simulink model "OFDMmodel_synch"  (R2025b)
settings: Solver=VariableStepAuto  StartTime=0.0  StopTime=inf  RelTol=1e-3
values from neighbouring files (symbols this model uses):
  BandasG = NFFT/4-4    (= 12)    [InitOFDM.m]
  Carriers = 1:NFFT    [InitOFDM.m]
  CP = 16    [InitOFDM.m]    (also in OFDMwideband_BEM2D.m = 32)
  DataCarrierIn = Carriers    [InitOFDM.m]
  DataCarriers = numel(DataCarrierIn)    [InitOFDM.m]
  DataCarriersFrame = DataCarriers*FrameSize    [InitOFDM.m]
  FrameSize = 40    [InitOFDM.m]
  FrameTime = Tsymbol*(FrameSize+2)    (= 0.000168)    [InitOFDM.m]
  NFFT = 64    [InitOFDM.m]    (also in OFDMwideband_BEM2D.m = 256)
  pilots = randsrc(numel(PilotIndex),1,[-1 1 1i 1i])*.71    [InitOFDM.m]
  PreambuloFrec = zeros(64,1)    [InitOFDM.m]    (also in Preambulo.mat = [0 0 0 0 0 0 0 0 4 0 0 0 ... (64 elements, 64x1)])
  Ts = 1/Fs    (= 5e-08)    [InitOFDM.m]    (also in OFDMwideband_BEM2D.m = 1e-07)
undefined symbols (not defined in the file or in its folder): ifftshift, j, jet, LogicIndex, Low, magnitude
libraries: simulink x9, dspsigops x7, dspxfrm3 x4, commrflib2 x3, dspswit3 x3, commchan3 x1, commofdm x1, dspobslib x1, dspmathops x1, commrandsrc3 x1, commdigbbndam3 x1
settings Model: PacingRate=0.001000  Creator=Fernando  LastModifiedBy=kutsari
settings SolverCC: AlgebraicLoopSolver=TrustRegion
settings DataIOCC: LimitDataPoints=on  MaxDataPoints=1  DSMLogging=off  SaveTime=off
settings DebuggingCC: SignalRangeChecking=warning  UnconnectedInputMsg=warning  UnconnectedOutputMsg=warning  UnconnectedLineMsg=warning  ArithmeticOperatorsInVariantConditions=warning
settings ModelReferenceCC: EnableRefExpFcnMdlSchedulingChecks=on
settings SFSimCC: CustomCodeUndefinedFunction=UseInterfaceOnly
settings RTWCC: GPUComputeCapability=3.5  DLArmComputeVersion=19.05

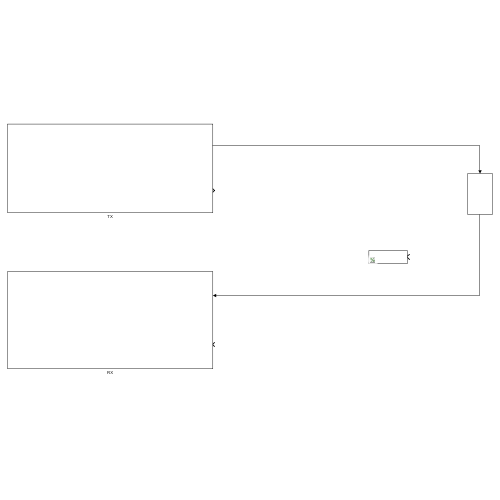
[thumbnail: Simulink's stored preview of the top-level diagram]
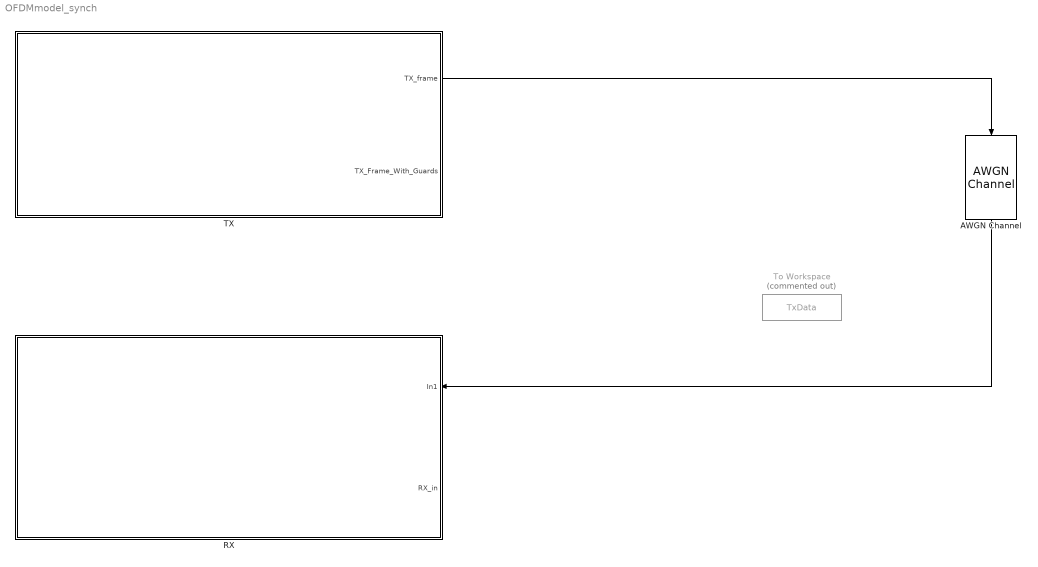
== system OFDMmodel_synch ==
  AWGN Channel : commchan3/AWGN Channel  LegacyMode=on  NoiseMethod="Signal to noise ratio  (SNR)"  noiseMode="Signal to noise ratio  (SNR)"  EbNo=10  EsNo=10  SNR=SNRdb  BitsPerSymbol=1  SignalPower=1  SpecifySymbolPeriod=off  SamplesPerSymbol=1  SymbolPeriod=1  VarianceSource=Parameter  Variance=1  RandomStream=Global stream  Seed=67  SimulateUsing=Code generation
  RX : Subsystem
  TX : Subsystem
  To Workspace : ToWorkspace  Commented=on  VariableName=TxData  SampleTime=-1
  wires:
  AWGN Channel/1 -> RX/1(In1)
  TX/1(TX_frame) -> AWGN Channel/1

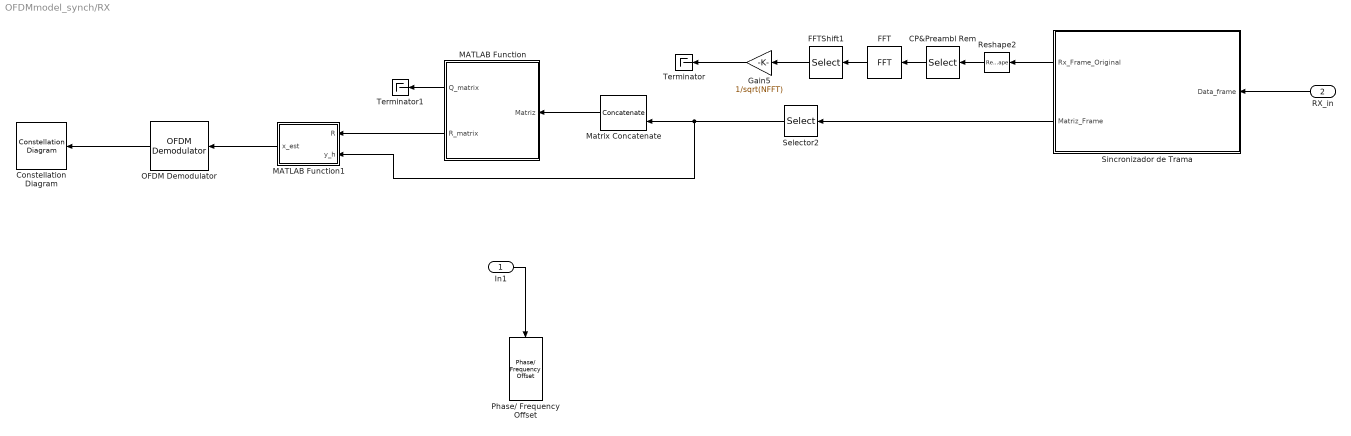
== system OFDMmodel_synch/RX ==
  In1 : Inport
  RX_in : Inport  Port=2
  CP&Preambl Rem : Selector  NumberOfDimensions=2  InputPortWidth=NFFT+CP  IndexOptions=Starting index (dialog),Starting index (dialog)  Indices=CP+1,2  OutputSizes=NFFT,FrameSize
  Constellation Diagram : ConstellationDiagram  DefaultConfigurationName=comm.scopes.ConstellationDiagramBlockCfg
  FFT : dspxfrm3/FFT  FFTImplementation=Auto  CompMethod=Table lookup  TableOpt=NEW  TableOptActive=Speed  BitRevOrder=off  Normalize=off  InheritFFTLength=on  FFTLength=64  WrapInput=on  roundingMode=Floor  overflowMode=off  firstCoeffDataTypeStr=Inherit: Same word length as input  firstCoeffLastDataTypeStr=Inherit: Same word length as input  outputMin=[]  outputMax=[]
  FFTShift1 : Selector  NumberOfDimensions=2  InputPortWidth=NFFT  IndexOptions=Index vector (dialog),Select all  Indices=ifftshift(Carriers),1  OutputSizes=1,1
  Gain5 : Gain  Gain=1/sqrt(NFFT)
  MATLAB Function : MATLAB Function  TreatAsAtomicUnit=on
  MATLAB Function1 : MATLAB Function  TreatAsAtomicUnit=on
  Matrix Concatenate : Concatenate  Mode=Multidimensional array  ConcatenateDimension=2
  OFDM Demodulator : commofdm/OFDM Demodulator  StatePerturbationForJacobian=1.0e-05  FFTLength=64  NumGuardBandCarriers=[6; 5]  RemoveDCCarrier=off  PilotOutputPort=off  PilotCarrierIndices=[12; 26; 40; 54]  CyclicPrefixLength=16  OversamplingFactor=1  NumSymbols=1  NumReceiveAntennas=1  SimulateUsing=Interpreted execution
  Phase/ Frequency Offset : commrflib2/Phase// Frequency Offset  phaseOffset=0  freqPort=off  freqOffset=5e3
  Reshape2 : Reshape  OutputDimensionality=Customize  OutputDimensions=[NFFT+CP,FrameSize+2]
  Selector2 : Selector  NumberOfDimensions=2  InputPortWidth=NFFT  IndexOptions=Index vector (dialog),Index vector (dialog)  Indices=DataCarrierIn,1  OutputSizes=1,1
  Sincronizador de Trama : Subsystem
  Terminator : Terminator
  Terminator1 : Terminator
  wires:
  Selector2/1 -> MATLAB Function1/2(y_h), Matrix Concatenate/2
  FFT/1 -> FFTShift1/1
  Sincronizador de Trama/2(Matriz_Frame) -> Selector2/1
  FFTShift1/1 -> Gain5/1
  Matrix Concatenate/1 -> MATLAB Function/1(Matriz)
  Reshape2/1 -> CP&Preambl Rem/1
  In1/1 -> Phase/ Frequency Offset/1
  Sincronizador de Trama/1(Rx_Frame_Original) -> Reshape2/1
  Gain5/1 -> Terminator/1
  MATLAB Function/1(Q_matrix) -> Terminator1/1
  CP&Preambl Rem/1 -> FFT/1
  MATLAB Function/2(R_matrix) -> MATLAB Function1/1(R)
  MATLAB Function1/1(x_est) -> OFDM Demodulator/1
  OFDM Demodulator/1 -> Constellation Diagram/1
  RX_in/1 -> Sincronizador de Trama/1(Data_frame)

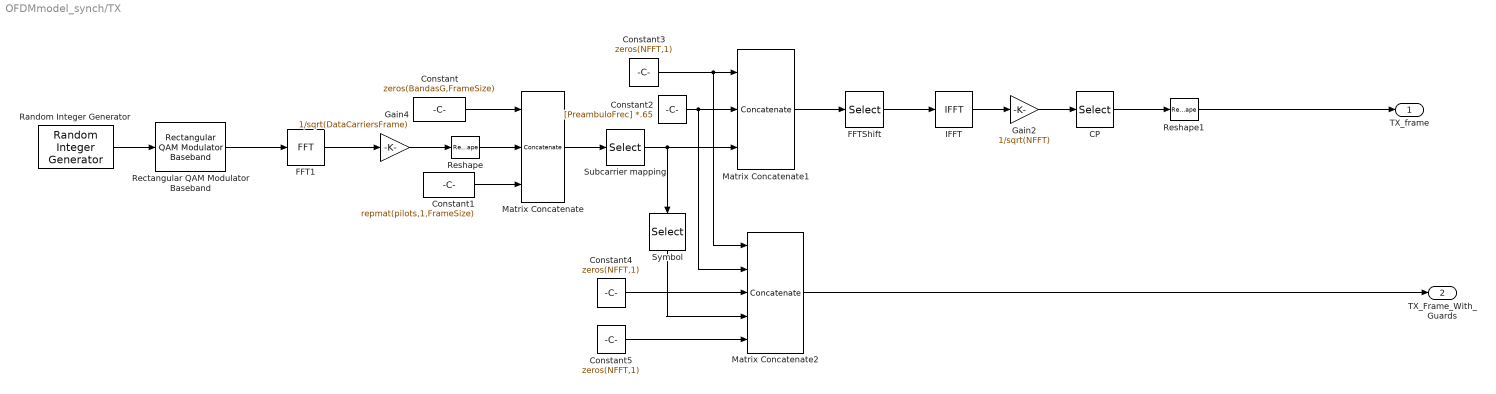
== system OFDMmodel_synch/TX ==
  CP : Selector  NumberOfDimensions=2  InputPortWidth=NFFT  IndexOptions=Index vector (dialog),Select all  Indices=[NFFT-CP+1:NFFT 1:NFFT],1  OutputSizes=1,1
  Constant : Constant  Value=zeros(BandasG,FrameSize)  VectorParams1D=off
  Constant1 : Constant  Value=repmat(pilots,1,FrameSize)  VectorParams1D=off
  Constant2 : Constant  Value=[PreambuloFrec] *.65  VectorParams1D=off
  Constant3 : Constant  Value=zeros(NFFT,1)  VectorParams1D=off
  Constant4 : Constant  Value=zeros(NFFT,1)  VectorParams1D=off
  Constant5 : Constant  Value=zeros(NFFT,1)  VectorParams1D=off
  FFT1 : dspxfrm3/FFT  FFTImplementation=Auto  CompMethod=Table lookup  TableOpt=NEW  TableOptActive=Speed  BitRevOrder=off  Normalize=off  InheritFFTLength=on  FFTLength=64  WrapInput=on  roundingMode=Floor  overflowMode=off  firstCoeffDataTypeStr=Inherit: Same word length as input  firstCoeffLastDataTypeStr=Inherit: Same word length as input  outputMin=[]  outputMax=[]
  FFTShift : Selector  NumberOfDimensions=2  InputPortWidth=NFFT  IndexOptions=Index vector (dialog),Select all  Indices=ifftshift(Carriers),1  OutputSizes=1,1
  Gain2 : Gain  Gain=1/sqrt(NFFT)
  Gain4 : Gain  Gain=1/sqrt(DataCarriersFrame)
  IFFT : dspxfrm3/IFFT  FFTImplementation=Auto  CompMethod=Table lookup  TableOpt=NEW  TableOptActive=Speed  BitRevOrder=off  cs_in=off  Normalize=off  InheritFFTLength=on  FFTLength=64  WrapInput=on  mode=Complex  outSamplingMode=Sample based  roundingMode=Floor  overflowMode=off  firstCoeffDataTypeStr=Inherit: Same word length as input  firstCoeffLastDataTypeStr=Inherit: Same word length as input  outputMin=[]  outputMax=[]
  Matrix Concatenate : Concatenate  NumInputs=3  Mode=Multidimensional array
  Matrix Concatenate1 : Concatenate  NumInputs=3  Mode=Multidimensional array  ConcatenateDimension=2
  Matrix Concatenate2 : Concatenate  NumInputs=5  Mode=Multidimensional array  ConcatenateDimension=2
  Random Integer Generator : commrandsrc3/Random Integer Generator  SetSize=ConstSize  SeedSource=Auto  Seed=0  SampleTime=FrameTime/(DataCarriers*FrameSize)  SamplesPerFrame=DataCarriers*FrameSize  OutputDataType=double  SimulateUsing=Interpreted execution
  Rectangular QAM Modulator Baseband : commdigbbndam3/Rectangular QAM Modulator Baseband  M=ConstSize  InType=Integer  Enc=Gray  Mapping=[0:15]  PowType=Average Power  MinDist=2  AvgPow=1  PeakPow=1  Ph=0  outDtype=double  outWordLen=16  outUDDataType=sfix(16)  outFracLenMode=Best precision  outFracLen=15  outDataTypeStr=double  outLastDataTypeStr=double
  Reshape : Reshape  OutputDimensionality=Customize  OutputDimensions=[DataCarriers,FrameSize]
  Reshape1 : Reshape  OutputDimensionality=Column vector (2-D)  OutputDimensions=[DataCarriers,FrameSize]
  Subcarrier mapping : Selector  NumberOfDimensions=2  InputPortWidth=NFFT  IndexOptions=Index vector (dialog),Select all  Indices=LogicIndex,1  OutputSizes=1,1
  Symbol : Selector  NumberOfDimensions=2  InputPortWidth=NFFT+CP  IndexOptions=Select all,Starting index (dialog)  Indices=CP+1,2  OutputSizes=NFFT,FrameSize-2
  TX_frame : Outport
  TX_Frame_With_Guards : Outport  Port=2
  wires:
  Rectangular QAM Modulator Baseband/1 -> FFT1/1
  CP/1 -> Reshape1/1
  Constant3/1 -> Matrix Concatenate2/1, Matrix Concatenate1/1
  Matrix Concatenate2/1 -> TX_Frame_With_Guards/1
  Matrix Concatenate/1 -> Subcarrier mapping/1
  Random Integer Generator/1 -> Rectangular QAM Modulator Baseband/1
  IFFT/1 -> Gain2/1
  FFT1/1 -> Gain4/1
  Gain4/1 -> Reshape/1
  Constant2/1 -> Matrix Concatenate2/2, Matrix Concatenate1/2
  Reshape/1 -> Matrix Concatenate/2
  Constant/1 -> Matrix Concatenate/1
  Gain2/1 -> CP/1
  Constant4/1 -> Matrix Concatenate2/3
  Subcarrier mapping/1 -> Matrix Concatenate1/3, Symbol/1
  Constant5/1 -> Matrix Concatenate2/5
  Constant1/1 -> Matrix Concatenate/3
  Symbol/1 -> Matrix Concatenate2/4
  Matrix Concatenate1/1 -> FFTShift/1
  FFTShift/1 -> IFFT/1
  Reshape1/1 -> TX_frame/1

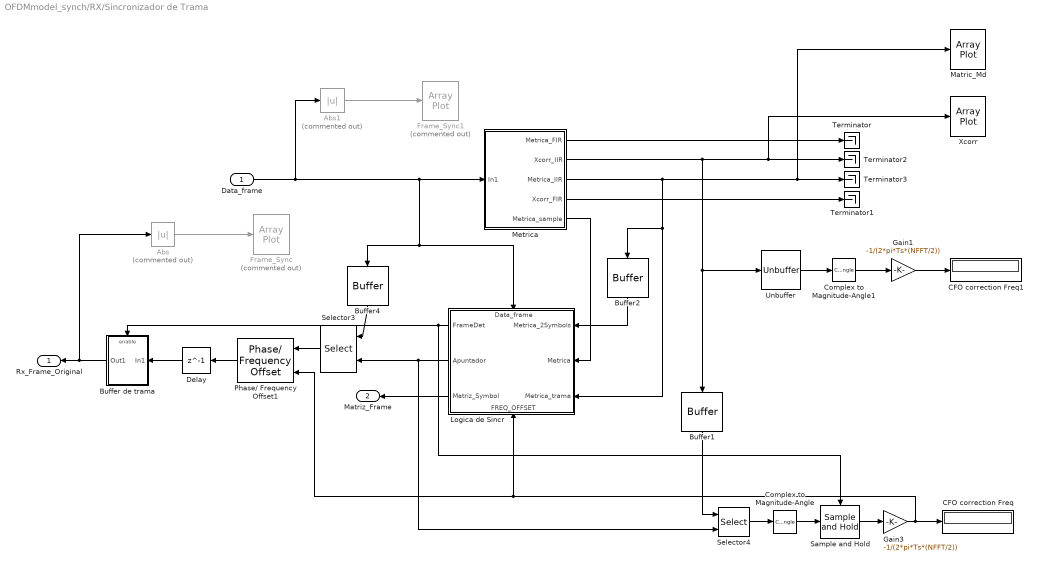
== system OFDMmodel_synch/RX/Sincronizador de Trama ==
  Data_frame : Inport
  Abs : Abs  Commented=on  SaturateOnIntegerOverflow=off
  Abs1 : Abs  Commented=on  SaturateOnIntegerOverflow=off
  Buffer de trama : Subsystem
  Buffer1 : Buffer  N=2*(NFFT+CP)  V=NFFT+CP  OutputFrames=off
  Buffer2 : Buffer  N=2*(NFFT+CP)  V=NFFT+CP  OutputFrames=off
  Buffer4 : Buffer  N=3*(NFFT+CP)  V=2*(NFFT+CP)  OutputFrames=off
  CFO correction Freq : Display
  CFO correction Freq1 : Display
  Complex to Magnitude-Angle : ComplexToMagnitudeAngle  Output=Angle
  Complex to Magnitude-Angle1 : ComplexToMagnitudeAngle  Output=Angle
  Delay : Delay  DelayLength=1
  Frame_Sync : ArrayPlot  Commented=on  WindowPosition=[1 41 1920 963]  AxesScaling=Manual  YLimits=[-0.276842,2.60957]  ShowGrid=off  ChannelNames="[\"\"]"  DefaultConfigurationName=dsp.scopes.ArrayPlotBlockSpecification
  Frame_Sync1 : ArrayPlot  Commented=on  WindowPosition=[1 41 1920 963]  AxesScaling=Manual  YLimits=[-0.026237,2.10871]  ShowGrid=off  ChannelNames="[\"\"]"  DefaultConfigurationName=dsp.scopes.ArrayPlotBlockSpecification
  Gain1 : Gain  Gain=-1/(2*pi*Ts*(NFFT/2))
  Gain3 : Gain  Gain=-1/(2*pi*Ts*(NFFT/2))
  Logica de Sincr : Subsystem
      settings: PortSchema="{\"entries\":[{\"content\":{\"sides\":[{\"content\":{\"connectorIds\":[\"In1\",\"In2\",\"In3\"]},\"type\":\"ConnectorPlacement.EquallySpacedRectSide\",\"uuid\":\"5f8267a0-6860-401f-8e05-bbfffcd5964b\"},{\"content\":{\"connectorIds\":[\"Out1\",\"Out2\",\"Out3\"],\"side\":\"RIGHT\"},\"type\":\"ConnectorPlacement.EquallySpacedRectSide\",\"uuid\":\"fea28aec-daf6-4e63-9655-5b68affc5124\"},{\"content\":{\"connectorIds\":[\"In4\"],\"side\":\"TOP\"},\"type\":\"ConnectorPlacement.EquallySpacedRectSide\",\"uuid\":\"72f5d6e1-ce9a-4296-9270-866e7a0a9494\"},{\"content\":{\"connectorIds\":[\"In5\"],\"side\":\"BOTTOM\"},\"type\":\"ConnectorPlacement.EquallySpacedRectSide\",\"uuid\":\"1736f37f-6e2b-4d11-abf7-aeb554299ece\"},{\"content\":{\"connectorIds\":[],\"side\":\"HIDDEN\"},\"type\":\"ConnectorPlacement.EquallySpacedRectSide\",\"uuid\":\"c53868b6-b813-45ed-ac94-1581b09a364c\"}]},\"type\":\"ConnectorPlacement.EquallySpacedConnector\",\"uuid\":\"ad7f4edf-12d2-4e3f-b534-0670d62195e0\"}],\"packageUris\":[\"http://schema.mathworks.com/mf0/Connector/R2020b\"],\"version\":\"1.0\"}"
  Matric_Md : ArrayPlot  WindowPosition=[481 42 958 954]  AxesScaling=Manual  YLimits=[-0.125,1.125]  ShowGrid=off  ChannelNames="[\"\"]"  DefaultConfigurationName=dsp.scopes.ArrayPlotBlockSpecification
  Metrica : Subsystem
  Phase/ Frequency Offset1 : commrflib2/Phase// Frequency Offset  phaseOffset=0  freqPort=on  freqOffset=16e3
  Sample and Hold : dspsigops/Sample and Hold  trig=Rising edge  initCond=0  latchinput=off
  Selector3 : Selector  InputPortWidth=3*(NFFT+CP)  IndexOptions=Starting index (port)  Indices=[1 3]  OutputSizes=NFFT+CP
  Selector4 : Selector  InputPortWidth=2*(NFFT+CP)  IndexOptions=Index vector (port)  Indices=[1 3]  OutputSizes=1
  Terminator{,1..3} (4 alike) : Terminator
  Unbuffer : Unbuffer
  Xcorr : ArrayPlot  WindowPosition=[481 42 958 954]  AxesScaling=Manual  YLimits=[-0.125,1.125]  ShowGrid=off  ChannelNames="[\"\"]"  DefaultConfigurationName=dsp.scopes.ArrayPlotBlockSpecification
  Rx_Frame_Original : Outport
  Matriz_Frame : Outport  Port=2
  wires:
  Phase/ Frequency Offset1/1 -> Delay/1
  Gain3/1 -> Logica de Sincr/5(FREQ_OFFSET), Phase/ Frequency Offset1/2, CFO correction Freq/1
  Buffer1/1 -> Selector4/1
  Logica de Sincr/2(Apuntador) -> Selector4/2, Selector3/2
  Sample and Hold/1 -> Gain3/1
  Logica de Sincr/1(FrameDet) -> Sample and Hold/Trigger, Buffer de trama/Enable
  Buffer4/1 -> Selector3/1
  Buffer2/1 -> Logica de Sincr/1(Metrica_2Symbols)
  Complex to Magnitude-Angle/1 -> Sample and Hold/1
  Selector3/1 -> Phase/ Frequency Offset1/1
  Metrica/2(Xcorr_IIR) -> Buffer1/1, Unbuffer/1, Xcorr/1, Terminator2/1
  Delay/1 -> Buffer de trama/1(In1)
  Selector4/1 -> Complex to Magnitude-Angle/1
  Data_frame/1 -> Abs1/1, Metrica/1(In1), Logica de Sincr/4(Data_frame), Buffer4/1
  Metrica/3(Metrica_IIR) -> Matric_Md/1, Terminator3/1, Buffer2/1, Logica de Sincr/3(Metrica_trama)
  Buffer de trama/1(Out1) -> Abs/1, Rx_Frame_Original/1
  Metrica/1(Metrica_FIR) -> Terminator/1
  Metrica/5(Metrica_sample) -> Logica de Sincr/2(Metrica)
  Abs/1 -> Frame_Sync/1
  Abs1/1 -> Frame_Sync1/1
  Logica de Sincr/3(Matriz_Symbol) -> Matriz_Frame/1
  Complex to Magnitude-Angle1/1 -> Gain1/1
  Gain1/1 -> CFO correction Freq1/1
  Unbuffer/1 -> Complex to Magnitude-Angle1/1
  Metrica/4(Xcorr_FIR) -> Terminator1/1

== system OFDMmodel_synch/RX/Sincronizador de Trama/Buffer de trama ==
  In1 : Inport
  Enable : EnablePort  ZeroCross=off
  Buffer5 : Buffer  N=(NFFT+CP)*(FrameSize+2)  OutputFrames=off
  Out1 : Outport
  wires:
  In1/1 -> Buffer5/1
  Buffer5/1 -> Out1/1

== system OFDMmodel_synch/RX/Sincronizador de Trama/Logica de Sincr ==
  Metrica_2Symbols : Inport
  Metrica : Inport  Port=2
  Metrica_trama : Inport  Port=3
  Data_frame : Inport  Port=4
  FREQ_OFFSET : Inport  Port=5
  Calculo_indice_Gonzalo_v1 : Subsystem
  Calculo_indice_Gonzalo_v2 : Subsystem
  Calculo_indice_Peña : Subsystem
  Display1 : Display
  Display4 : Display
  Terminator : Terminator
  Terminator1 : Terminator
  FrameDet : Outport
  Apuntador : Outport  Port=2
  Matriz_Symbol : Outport  Port=3
  wires:
  Metrica/1 -> Calculo_indice_Gonzalo_v2/1(Metrica), Calculo_indice_Gonzalo_v1/1(Trigger)
  Data_frame/1 -> Calculo_indice_Gonzalo_v2/2(Data_frame)
  FREQ_OFFSET/1 -> Calculo_indice_Gonzalo_v2/3(Freq_Offset)
  Calculo_indice_Gonzalo_v2/1(Matriz_Symbol) -> Matriz_Symbol/1
  Calculo_indice_Gonzalo_v1/1(Out1) -> Apuntador/1, Display4/1
  Metrica_trama/1 -> Calculo_indice_Gonzalo_v1/2(In2)
  Metrica_2Symbols/1 -> Calculo_indice_Peña/1(In1)
  Calculo_indice_Peña/1(Out1) -> Terminator/1
  Calculo_indice_Peña/2(Out2) -> FrameDet/1
  Calculo_indice_Gonzalo_v2/2(Apuntador_v2) -> Display1/1, Terminator1/1

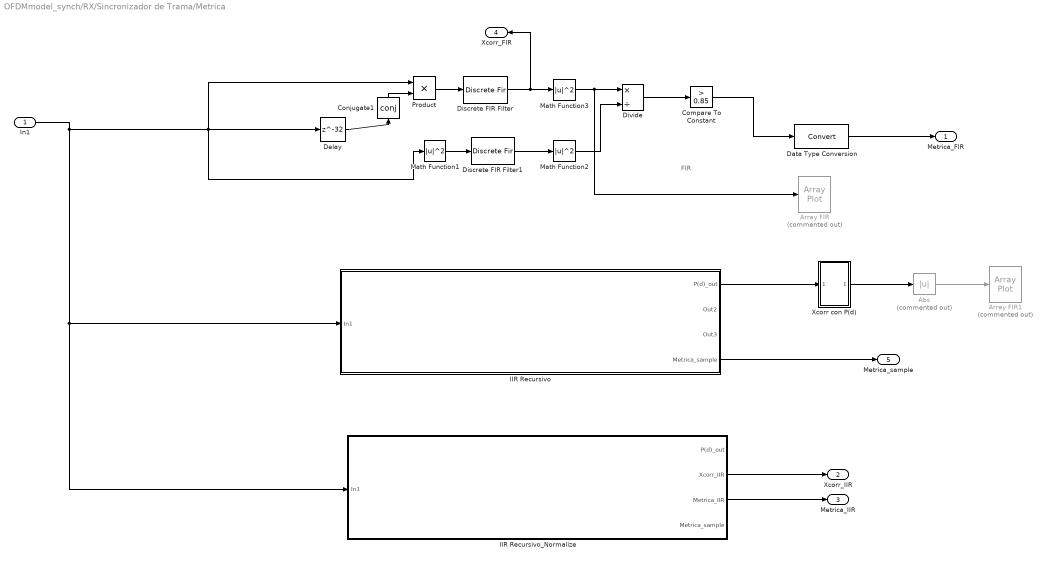
== system OFDMmodel_synch/RX/Sincronizador de Trama/Metrica ==
  note: FIR
  In1 : Inport
  Abs : Abs  Commented=on  SaturateOnIntegerOverflow=off
  Array FIR : ArrayPlot  Commented=on  WindowPosition=[480 -51 958 954]  AxesScaling=Manual  YLimits=[-821.624,7394.62]  ShowGrid=off  ChannelNames="[\"\"]"  DefaultConfigurationName=dsp.scopes.ArrayPlotBlockSpecification
  Array FIR1 : ArrayPlot  Commented=on  WindowPosition=[2 -5 1920 963]  AxesScaling=Manual  YLimits=[-16377.7,109222]  ShowGrid=off  ChannelNames="[\"\"]"  DefaultConfigurationName=dsp.scopes.ArrayPlotBlockSpecification
  Compare To Constant : simulink/Logic and Bit Operations/Compare To Constant  relop=>  const=0.85  OutDataTypeStr=uint8  ZeroCross=off
  Conjugate1 : Math  Operator=conj  SignedPower=on  RndMeth=Zero
  Data Type Conversion : DataTypeConversion  SaturateOnIntegerOverflow=off  RndMeth=Floor
  Delay : Delay  DelayLength=32  InputProcessing=Columns as channels (frame based)
  Discrete FIR Filter : DiscreteFir  Coefficients=ones(1,32)  InputProcessing=Columns as channels (frame based)
  Discrete FIR Filter1 : DiscreteFir  Coefficients=0.5*ones(1,NFFT)  InputProcessing=Columns as channels (frame based)
  Divide : Product  Inputs=*/
  IIR Recursivo : Subsystem
  IIR Recursivo_Normalize : Subsystem
  Math Function1 : Math  Operator=magnitude^2  SignedPower=on
  Math Function2 : Math  Operator=magnitude^2  SignedPower=on
  Math Function3 : Math  Operator=magnitude^2  SignedPower=on
  Product : Product
  Xcorr con P(d) : Subsystem
  Metrica_FIR : Outport
  Xcorr_IIR : Outport  Port=2
  Metrica_IIR : Outport  Port=3
  Xcorr_FIR : Outport  Port=4
  Metrica_sample : Outport  Port=5
  wires:
  Delay/1 -> Conjugate1/1
  Discrete FIR Filter/1 -> Xcorr_FIR/1, Math Function3/1
  Product/1 -> Discrete FIR Filter/1
  Math Function1/1 -> Discrete FIR Filter1/1
  Compare To Constant/1 -> Data Type Conversion/1
  Discrete FIR Filter1/1 -> Math Function2/1
  Math Function3/1 -> Array FIR/1, Divide/1
  Math Function2/1 -> Divide/2
  Data Type Conversion/1 -> Metrica_FIR/1
  Conjugate1/1 -> Product/2
  Divide/1 -> Compare To Constant/1
  In1/1 -> IIR Recursivo_Normalize/1(In1), IIR Recursivo/1(In1), Product/1, Delay/1, Math Function1/1
  IIR Recursivo/1(P(d)_out) -> Xcorr con P(d)/1(In1)
  Xcorr con P(d)/1(Out1) -> Abs/1
  Abs/1 -> Array FIR1/1
  IIR Recursivo/4(Metrica_sample) -> Metrica_sample/1
  IIR Recursivo_Normalize/2(Xcorr_IIR) -> Xcorr_IIR/1
  IIR Recursivo_Normalize/3(Metrica_IIR) -> Metrica_IIR/1

== system OFDMmodel_synch/RX/Sincronizador de Trama/Logica de Sincr/Calculo_indice_Gonzalo_v1 ==
  Trigger : Inport
  In2 : Inport  Port=2
  Bias1 : Bias  Bias=4  SaturateOnIntegerOverflow=off
  Compare To Constant : simulink/Logic and Bit Operations/Compare To Constant  relop=>=  const=NFFT+CP  OutDataTypeStr=boolean
  Display : Display
  Display1 : Display
  Gain : Gain  Gain=1/2
  Gain1 : Gain  Gain=transpose(1:42*(NFFT+CP))
  Rate Transition : RateTransition  OutPortSampleTime=4e-6
  Round1 : Rounding  Operator=round
  Sample and Hold1 : dspsigops/Sample and Hold  trig=Falling edge  initCond=0  latchinput=off
  Sample and Hold2 : dspsigops/Sample and Hold  trig=Rising edge  initCond=0  latchinput=off
  Sample and Hold3 : dspsigops/Sample and Hold  trig=Rising edge  initCond=0  latchinput=off
  Saturation1 : Saturate  UpperLimit=2*(NFFT+CP)+1  LowerLimit=1
  Sum2 : Sum
  Unbuffer : Unbuffer
  Out1 : Outport
  wires:
  Unbuffer/1 -> Sample and Hold1/1, Sample and Hold2/1
  Sample and Hold1/1 -> Sum2/2, Display1/1
  Sample and Hold2/1 -> Sum2/1, Display/1
  Gain/1 -> Round1/1
  Sample and Hold3/1 -> Bias1/1
  Compare To Constant/1 -> Sample and Hold3/Trigger
  Bias1/1 -> Saturation1/1
  Sum2/1 -> Gain/1
  Saturation1/1 -> Rate Transition/1
  Trigger/1 -> Sample and Hold2/Trigger, Sample and Hold1/Trigger
  Round1/1 -> Compare To Constant/1, Sample and Hold3/1
  In2/1 -> Gain1/1
  Gain1/1 -> Unbuffer/1
  Rate Transition/1 -> Out1/1

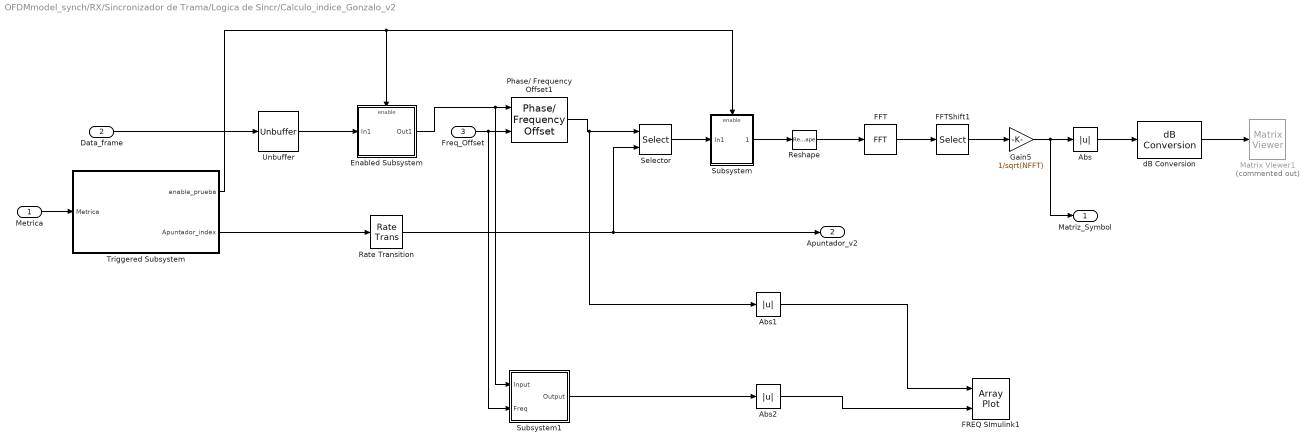
== system OFDMmodel_synch/RX/Sincronizador de Trama/Logica de Sincr/Calculo_indice_Gonzalo_v2 ==
  Metrica : Inport
  Data_frame : Inport  Port=2
  Freq_Offset : Inport  Port=3
  Abs : Abs  SaturateOnIntegerOverflow=off
  Abs1 : Abs  SaturateOnIntegerOverflow=off
  Abs2 : Abs  SaturateOnIntegerOverflow=off
  Enabled Subsystem : Subsystem  TreatAsAtomicUnit=on
  FFT : dspxfrm3/FFT  FFTImplementation=Auto  CompMethod=Table lookup  TableOpt=NEW  TableOptActive=Speed  BitRevOrder=off  Normalize=off  InheritFFTLength=on  FFTLength=64  WrapInput=on  roundingMode=Floor  overflowMode=off  firstCoeffDataTypeStr=Inherit: Same word length as input  firstCoeffLastDataTypeStr=Inherit: Same word length as input  outputMin=[]  outputMax=[]
  FFTShift1 : Selector  NumberOfDimensions=2  InputPortWidth=NFFT  IndexOptions=Index vector (dialog),Select all  Indices=ifftshift(Carriers),1  OutputSizes=1,1
  FREQ SImulink1 : ArrayPlot  NumInputPorts=2  WindowPosition=[99.000000,117.000000,1918.000000,954.000000,]  ScopeFrameLocation=window  AxesScaling=Manual  YLimits=[-0.0514301,1.04318]  ShowGrid=off  ChannelNames="[\"\"]"  DefaultConfigurationName=dsp.scopes.ArrayPlotBlockSpecification
  Gain5 : Gain  Gain=1/sqrt(NFFT)
  Matrix Viewer1 : dspobslib/Matrix Viewer  Commented=on  ImageParams=off  CMapStr=jet(256)  AxisColorbar=on  AxisParams=off  AxisOrigin=Upper left corner  AxisTickMode=Auto  XTickRange=[0 1]  YTickRange=[0 1]  XLabel=X-axis  YLabel=Y-axis  ZLabel=Z-axis  FigPos=[962 42 958 1008]  AxisZoom=off
      settings: YMin=-30  YMax=-20
  Phase/ Frequency Offset1 : commrflib2/Phase// Frequency Offset  phaseOffset=0  freqPort=on  freqOffset=16e3
  Rate Transition : RateTransition  OutPortSampleTime=4e-6
  Reshape : Reshape  OutputDimensionality=Customize  OutputDimensions=[(NFFT),40]
  Selector : Selector  InputPortWidth=NFFT+CP  IndexOptions=Starting index (port)  Indices=[1 3]  OutputSizes=NFFT
  Subsystem : Subsystem
  Subsystem1 : Subsystem
  Triggered Subsystem : Subsystem  TreatAsAtomicUnit=on
  Unbuffer : Unbuffer
  dB Conversion : dspmathops/dB Conversion  dBtype=dB  intype=Amplitude  R=1  fuzz=off
  Matriz_Symbol : Outport
  Apuntador_v2 : Outport  Port=2
  wires:
  Metrica/1 -> Triggered Subsystem/1(Metrica)
  Data_frame/1 -> Unbuffer/1
  Abs/1 -> dB Conversion/1
  Unbuffer/1 -> Enabled Subsystem/1(In1)
  Enabled Subsystem/1(Out1) -> Subsystem1/1(Input), Phase/ Frequency Offset1/1
  Rate Transition/1 -> Selector/2, Apuntador_v2/1
  dB Conversion/1 -> Matrix Viewer1/1
  FFT/1 -> FFTShift1/1
  FFTShift1/1 -> Gain5/1
  Reshape/1 -> FFT/1
  Gain5/1 -> Matriz_Symbol/1, Abs/1
  Subsystem/1(Trama_sin_CP) -> Reshape/1
  Phase/ Frequency Offset1/1 -> Abs1/1, Selector/1
  Freq_Offset/1 -> Subsystem1/2(Freq), Phase/ Frequency Offset1/2
  Selector/1 -> Subsystem/1(In1)
  Triggered Subsystem/2(Apuntador_index) -> Rate Transition/1
  Triggered Subsystem/1(enable_prueba) -> Subsystem/Enable, Enabled Subsystem/Enable
  Subsystem1/1(Output) -> Abs2/1
  Abs1/1 -> FREQ SImulink1/1
  Abs2/1 -> FREQ SImulink1/2

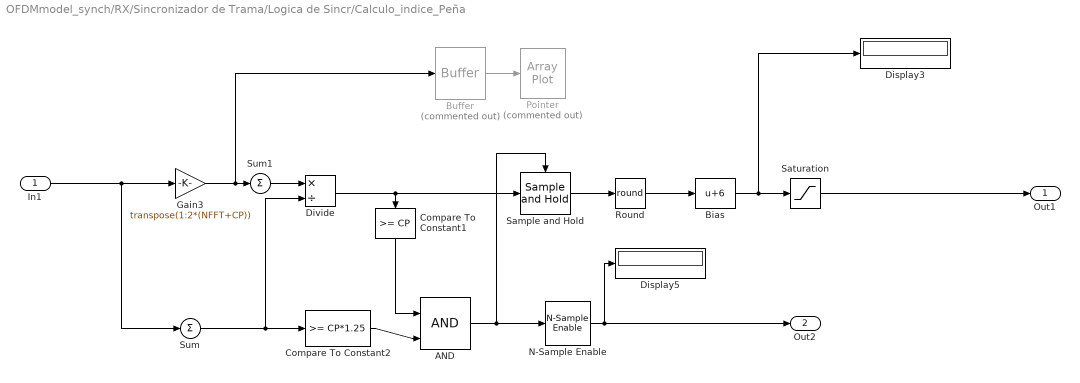
== system OFDMmodel_synch/RX/Sincronizador de Trama/Logica de Sincr/Calculo_indice_Peña ==
  In1 : Inport
  AND : Logic  IconShape=distinctive  AllPortsSameDT=off  OutDataTypeStr=boolean
  Bias : Bias  Bias=6  SaturateOnIntegerOverflow=off
  Buffer : Buffer  Commented=on  N=2*(NFFT + CP)  OutputFrames=off
  Compare To Constant1 : simulink/Logic and Bit Operations/Compare To Constant  relop=>=  const=CP  OutDataTypeStr=boolean  ZeroCross=off
  Compare To Constant2 : simulink/Logic and Bit Operations/Compare To Constant  relop=>=  const=CP*1.25  OutDataTypeStr=boolean  ZeroCross=off
  Display3 : Display
  Display5 : Display
  Divide : Product  Inputs=*/
  Gain3 : Gain  Gain=transpose(1:2*(NFFT+CP))
  N-Sample Enable : dspswit3/N-Sample Enable  N=FrameSize+1  ActiveLevel=Low (0)  reset=on  TriggerType=Rising edge  Ts=1  DataType=Logical
  Pointer : ArrayPlot  Commented=on  WindowPosition=[481 42 958 954]  AxesScaling=Manual  YLimits=[-16.5,168.5]  ShowGrid=off  ChannelNames="[\"\"]"  DefaultConfigurationName=dsp.scopes.ArrayPlotBlockSpecification
  Round : Rounding  Operator=round
  Sample and Hold : dspsigops/Sample and Hold  trig=Rising edge  initCond=0  latchinput=off
  Saturation : Saturate  UpperLimit=2*(NFFT+CP)+1  LowerLimit=1
  Sum : Sum  Inputs=+
  Sum1 : Sum  Inputs=+
  Out1 : Outport
  Out2 : Outport  Port=2
  wires:
  Sum/1 -> Divide/2, Compare To Constant2/1
  Bias/1 -> Display3/1, Saturation/1
  Gain3/1 -> Buffer/1, Sum1/1
  Sample and Hold/1 -> Round/1
  Divide/1 -> Sample and Hold/1, Compare To Constant1/1
  Compare To Constant2/1 -> AND/2
  Buffer/1 -> Pointer/1
  AND/1 -> Sample and Hold/Trigger, N-Sample Enable/1
  In1/1 -> Sum/1, Gain3/1
  N-Sample Enable/1 -> Out2/1, Display5/1
  Round/1 -> Bias/1
  Saturation/1 -> Out1/1
  Sum1/1 -> Divide/1
  Compare To Constant1/1 -> AND/1

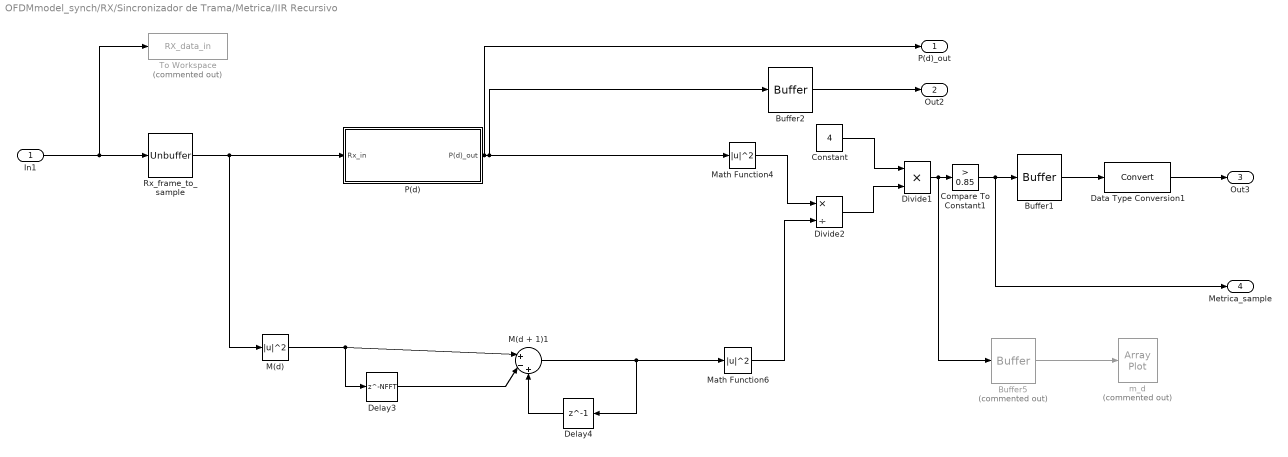
== system OFDMmodel_synch/RX/Sincronizador de Trama/Metrica/IIR Recursivo ==
  In1 : Inport
  Buffer1 : Buffer  N=(NFFT + CP) * 42  OutputFrames=off
  Buffer2 : Buffer  N=(NFFT + CP) * 42  OutputFrames=off
  Buffer5 : Buffer  Commented=on  N=(NFFT + CP) * 42  OutputFrames=off
  Compare To Constant1 : simulink/Logic and Bit Operations/Compare To Constant  relop=>  const=0.85  OutDataTypeStr=uint8  ZeroCross=off
  Constant : Constant  Value=4
  Data Type Conversion1 : DataTypeConversion  SaturateOnIntegerOverflow=off  RndMeth=Floor
  Delay3 : Delay  DelayLength=NFFT
  Delay4 : Delay  DelayLength=1
  Divide1 : Product  Inputs=**
  Divide2 : Product  Inputs=*/
  M(d + 1)1 : Sum  Inputs=|+-+
  M(d) : Math  Operator=magnitude^2  SignedPower=on
  Math Function4 : Math  Operator=magnitude^2  SignedPower=on
  Math Function6 : Math  Operator=magnitude^2  SignedPower=on
  P(d) : Subsystem
  Rx_frame_to_sample : Unbuffer
  To Workspace : ToWorkspace  Commented=on  VariableName=RX_data_in  SaveFormat=Timeseries  SampleTime=-1
  m_d : ArrayPlot  Commented=on  WindowPosition=[1 41 1920 963]  AxesScaling=Manual  YLimits=[-0.116212,1.04604]  ShowGrid=off  ChannelNames="[\"\"]"  DefaultConfigurationName=dsp.scopes.ArrayPlotBlockSpecification
  P(d)_out : Outport
  Out2 : Outport  Port=2
  Out3 : Outport  Port=3
  Metrica_sample : Outport  Port=4
  wires:
  M(d)/1 -> M(d + 1)1/1, Delay3/1
  Delay4/1 -> M(d + 1)1/3
  Buffer1/1 -> Data Type Conversion1/1
  Math Function6/1 -> Divide2/2
  Compare To Constant1/1 -> Metrica_sample/1, Buffer1/1
  Divide2/1 -> Divide1/2
  Divide1/1 -> Buffer5/1, Compare To Constant1/1
  Buffer2/1 -> Out2/1
  Delay3/1 -> M(d + 1)1/2
  Math Function4/1 -> Divide2/1
  Constant/1 -> Divide1/1
  In1/1 -> To Workspace/1, Rx_frame_to_sample/1
  Data Type Conversion1/1 -> Out3/1
  M(d + 1)1/1 -> Math Function6/1, Delay4/1
  Buffer5/1 -> m_d/1
  Rx_frame_to_sample/1 -> P(d)/1(Rx_in), M(d)/1
  P(d)/1(P(d)_out) -> P(d)_out/1, Buffer2/1, Math Function4/1

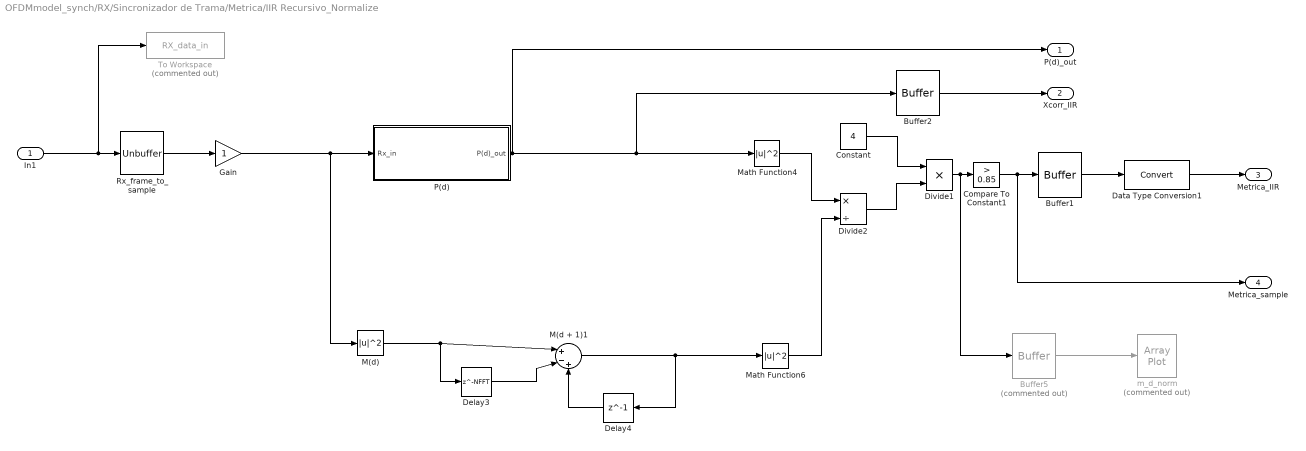
== system OFDMmodel_synch/RX/Sincronizador de Trama/Metrica/IIR Recursivo_Normalize ==
  In1 : Inport
  Buffer1 : Buffer  N=(NFFT + CP) * 42  OutputFrames=off
  Buffer2 : Buffer  N=(NFFT + CP) * 42  OutputFrames=off
  Buffer5 : Buffer  Commented=on  N=(NFFT + CP) * 42  OutputFrames=off
  Compare To Constant1 : simulink/Logic and Bit Operations/Compare To Constant  relop=>  const=0.85  OutDataTypeStr=uint8  ZeroCross=off
  Constant : Constant  Value=4
  Data Type Conversion1 : DataTypeConversion  SaturateOnIntegerOverflow=off  RndMeth=Floor
  Delay3 : Delay  DelayLength=NFFT
  Delay4 : Delay  DelayLength=1
  Divide1 : Product  Inputs=**
  Divide2 : Product  Inputs=*/
  Gain : Gain
  M(d + 1)1 : Sum  Inputs=|+-+
  M(d) : Math  Operator=magnitude^2  SignedPower=on
  Math Function4 : Math  Operator=magnitude^2  SignedPower=on
  Math Function6 : Math  Operator=magnitude^2  SignedPower=on
  P(d) : Subsystem
  Rx_frame_to_sample : Unbuffer
  To Workspace : ToWorkspace  Commented=on  VariableName=RX_data_in  SaveFormat=Timeseries  SampleTime=-1
  m_d_norm : ArrayPlot  Commented=on  WindowPosition=[1 41 1920 963]  AxesScaling=Manual  YLimits=[-0.116212,1.04604]  ShowGrid=off  ChannelNames="[\"\"]"  DefaultConfigurationName=dsp.scopes.ArrayPlotBlockSpecification
  P(d)_out : Outport
  Xcorr_IIR : Outport  Port=2
  Metrica_IIR : Outport  Port=3
  Metrica_sample : Outport  Port=4
  wires:
  P(d)/1(P(d)_out) -> Math Function4/1, Buffer2/1, P(d)_out/1
  Rx_frame_to_sample/1 -> Gain/1
  Buffer5/1 -> m_d_norm/1
  M(d + 1)1/1 -> Delay4/1, Math Function6/1
  Data Type Conversion1/1 -> Metrica_IIR/1
  In1/1 -> Rx_frame_to_sample/1, To Workspace/1
  Constant/1 -> Divide1/1
  Math Function4/1 -> Divide2/1
  Delay3/1 -> M(d + 1)1/2
  Buffer2/1 -> Xcorr_IIR/1
  Divide1/1 -> Compare To Constant1/1, Buffer5/1
  Divide2/1 -> Divide1/2
  Compare To Constant1/1 -> Buffer1/1, Metrica_sample/1
  Math Function6/1 -> Divide2/2
  Buffer1/1 -> Data Type Conversion1/1
  Delay4/1 -> M(d + 1)1/3
  M(d)/1 -> Delay3/1, M(d + 1)1/1
  Gain/1 -> P(d)/1(Rx_in), M(d)/1

== system OFDMmodel_synch/RX/Sincronizador de Trama/Metrica/Xcorr con P(d) ==
  In1 : Inport
  Buffer3 : Buffer  N=(NFFT + CP) * 42  OutputFrames=off
  Conjugate3 : Math  Operator=conj  SignedPower=on  RndMeth=Zero
  Delay1 : Delay  DelayLength=1
  Delay2 : Delay  DelayLength=NFFT/2  InputProcessing=Columns as channels (frame based)
  Delay5 : Delay  DelayLength=NFFT/2  InputProcessing=Columns as channels (frame based)
  P(d + 1) : Sum  Inputs=|+-+
  P(d) : Product
  Out1 : Outport
  wires:
  Conjugate3/1 -> P(d)/2
  P(d)/1 -> Delay2/1, P(d + 1)/1
  Delay2/1 -> P(d + 1)/2
  Delay5/1 -> Conjugate3/1
  Delay1/1 -> P(d + 1)/3
  In1/1 -> P(d)/1, Delay5/1
  Buffer3/1 -> Out1/1
  P(d + 1)/1 -> Delay1/1, Buffer3/1

== system OFDMmodel_synch/RX/Sincronizador de Trama/Logica de Sincr/Calculo_indice_Gonzalo_v2/Enabled Subsystem ==
  In1 : Inport
  Enable : EnablePort
  Buffer : Buffer  N=NFFT + CP  OutputFrames=off
  Out1 : Outport
  wires:
  In1/1 -> Buffer/1
  Buffer/1 -> Out1/1

== system OFDMmodel_synch/RX/Sincronizador de Trama/Logica de Sincr/Calculo_indice_Gonzalo_v2/Subsystem ==
  In1 : Inport
  Enable : EnablePort
  Buffer : Buffer  N=(NFFT) * 40  OutputFrames=off
  Trama_sin_CP : Outport
  wires:
  In1/1 -> Buffer/1
  Buffer/1 -> Trama_sin_CP/1

== system OFDMmodel_synch/RX/Sincronizador de Trama/Logica de Sincr/Calculo_indice_Gonzalo_v2/Subsystem1 ==
  Input : Inport
  Freq : Inport  Port=2
  Cosine : simulink/Lookup Tables/Cosine  Formula=exp(j*2*pi*u)  NumDataPoints=(2^5)+1  OutputWordLength=16  InternalRulePriority=Speed
  Product : Product
  Output : Outport
  wires:
  Freq/1 -> Cosine/1
  Cosine/1 -> Product/2
  Input/1 -> Product/1
  Product/1 -> Output/1

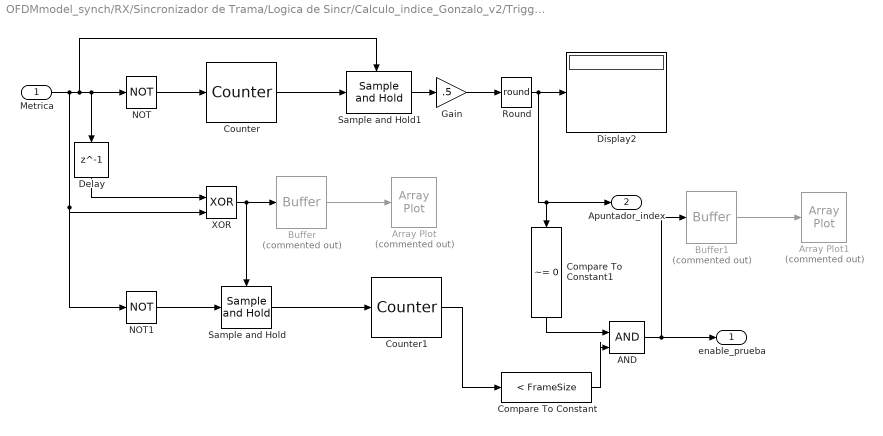
== system OFDMmodel_synch/RX/Sincronizador de Trama/Logica de Sincr/Calculo_indice_Gonzalo_v2/Triggered Subsystem ==
  Metrica : Inport
  AND : Logic  IconShape=distinctive  AllPortsSameDT=off  OutDataTypeStr=boolean
  Array Plot : ArrayPlot  Commented=on  WindowPosition=[2 42 1918 954]  Visible=on  AxesScaling=Manual  YLimits=[-0.0210134,1.03035]  ShowGrid=off  ChannelNames="[\"\"]"  DefaultConfigurationName=dsp.scopes.ArrayPlotBlockSpecification
  Array Plot1 : ArrayPlot  Commented=on  WindowPosition=[-1919 41 1920 963]  AxesScaling=Manual  YLimits=[-0.0584261,0.108841]  ShowGrid=off  ChannelNames="[\"\"]"  DefaultConfigurationName=dsp.scopes.ArrayPlotBlockSpecification
  Buffer : Buffer  Commented=on  N=(80*42)  OutputFrames=off
  Buffer1 : Buffer  Commented=on  N=(80*42)  OutputFrames=off
  Compare To Constant : simulink/Logic and Bit Operations/Compare To Constant  relop=<  const=FrameSize  OutDataTypeStr=boolean
  Compare To Constant1 : simulink/Logic and Bit Operations/Compare To Constant  relop=~=  const=0  OutDataTypeStr=boolean
  Counter : dspswit3/Counter  Direction=Up  CountEvent=Free running  CounterSize=User defined  MaxCount=79  InitialCount=1  Output=Count  HitValue=32  ResetInput=on  SamplesPerFrame=1  Ts=50e-9  CntDtype=double  HitDtype=Logical
  Counter1 : dspswit3/Counter  Direction=Up  CountEvent=Free running  CounterSize=User defined  MaxCount=79  InitialCount=0  Output=Count  HitValue=32  ResetInput=on  SamplesPerFrame=1  Ts=4e-6  CntDtype=double  HitDtype=Logical
  Delay : Delay  DelayLength=1
  Display2 : Display
  Gain : Gain  Gain=.5
  NOT : Logic  Operator=NOT  IconShape=distinctive  AllPortsSameDT=off  OutDataTypeStr=boolean
  NOT1 : Logic  Operator=NOT  IconShape=distinctive  AllPortsSameDT=off  OutDataTypeStr=boolean
  Round : Rounding  Operator=round
  Sample and Hold : dspsigops/Sample and Hold  trig=Rising edge  initCond=1  latchinput=on
  Sample and Hold1 : dspsigops/Sample and Hold  trig=Falling edge  initCond=1  latchinput=on
  XOR : Logic  Operator=XOR  IconShape=distinctive  AllPortsSameDT=off  OutDataTypeStr=boolean
  enable_prueba : Outport
  Apuntador_index : Outport  Port=2
  wires:
  Sample and Hold1/1 -> Gain/1
  Gain/1 -> Round/1
  Counter/1 -> Sample and Hold1/1
  Round/1 -> Compare To Constant1/1, Apuntador_index/1, Display2/1
  Metrica/1 -> NOT1/1, XOR/2, Sample and Hold1/Trigger, NOT/1, Delay/1
  NOT/1 -> Counter/1
  Delay/1 -> XOR/1
  Buffer/1 -> Array Plot/1
  XOR/1 -> Sample and Hold/Trigger, Buffer/1
  Counter1/1 -> Compare To Constant/1
  Sample and Hold/1 -> Counter1/1
  NOT1/1 -> Sample and Hold/1
  AND/1 -> Buffer1/1, enable_prueba/1
  Compare To Constant/1 -> AND/2
  Compare To Constant1/1 -> AND/1
  Buffer1/1 -> Array Plot1/1

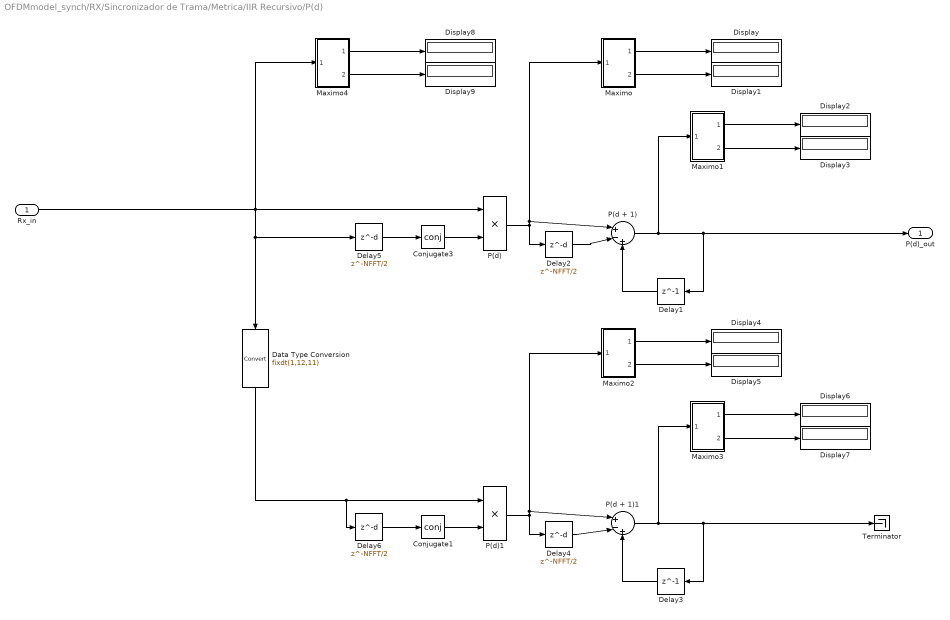
== system OFDMmodel_synch/RX/Sincronizador de Trama/Metrica/IIR Recursivo/P(d) ==
  Rx_in : Inport
  Conjugate1 : Math  Operator=conj  SignedPower=on  RndMeth=Zero
  Conjugate3 : Math  Operator=conj  SignedPower=on  RndMeth=Zero
  Data Type Conversion : DataTypeConversion  OutDataTypeStr=fixdt(1,12,11)  SaturateOnIntegerOverflow=off  RndMeth=Floor  LockScale=on
  Delay1 : Delay  DelayLength=1
  Delay{2,4..6} (4 alike) : Delay  DelayLength=NFFT/2  InputProcessing=Columns as channels (frame based)
  Delay3 : Delay  DelayLength=1
  Display{,1..9} (10 alike) : Display
  Maximo : Subsystem
  Maximo1 : Subsystem
  Maximo2 : Subsystem
  Maximo3 : Subsystem
  Maximo4 : Subsystem
  P(d + 1) : Sum  Inputs=|+-+
  P(d + 1)1 : Sum  Inputs=|+-+
  P(d) : Product
  P(d)1 : Product
  Terminator : Terminator
  P(d)_out : Outport
  wires:
  Delay2/1 -> P(d + 1)/2
  P(d)/1 -> Maximo/1(In1), P(d + 1)/1, Delay2/1
  Delay1/1 -> P(d + 1)/3
  Delay5/1 -> Conjugate3/1
  Conjugate3/1 -> P(d)/2
  P(d + 1)/1 -> Maximo1/1(In1), Delay1/1, P(d)_out/1
  Maximo/1(Real) -> Display/1
  Maximo/2(Imag) -> Display1/1
  Maximo1/2(Imag) -> Display3/1
  Maximo1/1(Real) -> Display2/1
  Maximo3/1(Real) -> Display6/1
  Maximo2/1(Real) -> Display4/1
  Maximo2/2(Imag) -> Display5/1
  Delay3/1 -> P(d + 1)1/3
  P(d)1/1 -> Maximo2/1(In1), P(d + 1)1/1, Delay4/1
  Delay4/1 -> P(d + 1)1/2
  Delay6/1 -> Conjugate1/1
  P(d + 1)1/1 -> Maximo3/1(In1), Terminator/1, Delay3/1
  Data Type Conversion/1 -> Delay6/1, P(d)1/1
  Maximo3/2(Imag) -> Display7/1
  Conjugate1/1 -> P(d)1/2
  Maximo4/2(Imag) -> Display9/1
  Maximo4/1(Real) -> Display8/1
  Rx_in/1 -> Maximo4/1(Rx_in), P(d)/1, Data Type Conversion/1, Delay5/1

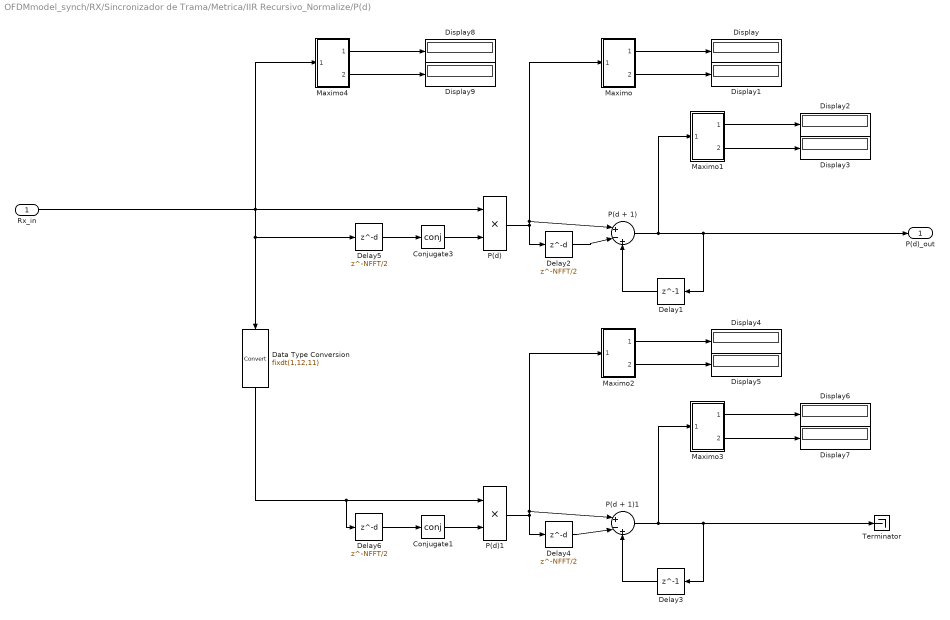
== system OFDMmodel_synch/RX/Sincronizador de Trama/Metrica/IIR Recursivo_Normalize/P(d) ==
  Rx_in : Inport
  Conjugate1 : Math  Operator=conj  SignedPower=on  RndMeth=Zero
  Conjugate3 : Math  Operator=conj  SignedPower=on  RndMeth=Zero
  Data Type Conversion : DataTypeConversion  OutDataTypeStr=fixdt(1,12,11)  SaturateOnIntegerOverflow=off  RndMeth=Floor  LockScale=on
  Delay1 : Delay  DelayLength=1
  Delay{2,4..6} (4 alike) : Delay  DelayLength=NFFT/2  InputProcessing=Columns as channels (frame based)
  Delay3 : Delay  DelayLength=1
  Display{,1..9} (10 alike) : Display
  Maximo : Subsystem
  Maximo1 : Subsystem
  Maximo2 : Subsystem
  Maximo3 : Subsystem
  Maximo4 : Subsystem
  P(d + 1) : Sum  Inputs=|+-+
  P(d + 1)1 : Sum  Inputs=|+-+
  P(d) : Product
  P(d)1 : Product
  Terminator : Terminator
  P(d)_out : Outport
  wires:
  Rx_in/1 -> Delay5/1, Data Type Conversion/1, P(d)/1, Maximo4/1(Rx_in)
  Maximo4/1(Real) -> Display8/1
  Maximo4/2(Imag) -> Display9/1
  Conjugate1/1 -> P(d)1/2
  Maximo3/2(Imag) -> Display7/1
  Data Type Conversion/1 -> P(d)1/1, Delay6/1
  P(d + 1)1/1 -> Delay3/1, Terminator/1, Maximo3/1(In1)
  Delay6/1 -> Conjugate1/1
  Delay4/1 -> P(d + 1)1/2
  P(d)1/1 -> Delay4/1, P(d + 1)1/1, Maximo2/1(In1)
  Delay3/1 -> P(d + 1)1/3
  Maximo2/2(Imag) -> Display5/1
  Maximo2/1(Real) -> Display4/1
  Maximo3/1(Real) -> Display6/1
  Maximo1/1(Real) -> Display2/1
  Maximo1/2(Imag) -> Display3/1
  Maximo/2(Imag) -> Display1/1
  Maximo/1(Real) -> Display/1
  P(d + 1)/1 -> P(d)_out/1, Delay1/1, Maximo1/1(In1)
  Conjugate3/1 -> P(d)/2
  Delay5/1 -> Conjugate3/1
  Delay1/1 -> P(d + 1)/3
  P(d)/1 -> Delay2/1, P(d + 1)/1, Maximo/1(In1)
  Delay2/1 -> P(d + 1)/2

== system OFDMmodel_synch/RX/Sincronizador de Trama/Metrica/IIR Recursivo/P(d)/Maximo ==
  In1 : Inport
  Abs : Abs  SaturateOnIntegerOverflow=off
  Abs1 : Abs  SaturateOnIntegerOverflow=off
  Complex to Real-Imag : ComplexToRealImag
  Delay : Delay  DelayLength=1
  Delay1 : Delay  DelayLength=1
  Max : MinMax  Function=max  Inputs=2
  Max1 : MinMax  Function=max  Inputs=2
  Real : Outport
  Imag : Outport  Port=2
  wires:
  Max/1 -> Real/1, Delay/1
  Delay/1 -> Max/1
  Max1/1 -> Imag/1, Delay1/1
  Delay1/1 -> Max1/1
  Complex to Real-Imag/2 -> Abs1/1
  Complex to Real-Imag/1 -> Abs/1
  In1/1 -> Complex to Real-Imag/1
  Abs/1 -> Max/2
  Abs1/1 -> Max1/2

== system OFDMmodel_synch/RX/Sincronizador de Trama/Metrica/IIR Recursivo/P(d)/Maximo1 ==
  In1 : Inport
  Abs : Abs  SaturateOnIntegerOverflow=off
  Abs1 : Abs  SaturateOnIntegerOverflow=off
  Complex to Real-Imag : ComplexToRealImag
  Delay : Delay  DelayLength=1
  Delay1 : Delay  DelayLength=1
  Max : MinMax  Function=max  Inputs=2
  Max1 : MinMax  Function=max  Inputs=2
  Real : Outport
  Imag : Outport  Port=2
  wires:
  Abs1/1 -> Max1/2
  Abs/1 -> Max/2
  In1/1 -> Complex to Real-Imag/1
  Complex to Real-Imag/1 -> Abs/1
  Complex to Real-Imag/2 -> Abs1/1
  Delay1/1 -> Max1/1
  Max1/1 -> Delay1/1, Imag/1
  Delay/1 -> Max/1
  Max/1 -> Delay/1, Real/1

== system OFDMmodel_synch/RX/Sincronizador de Trama/Metrica/IIR Recursivo/P(d)/Maximo2 ==
  In1 : Inport
  Abs : Abs  SaturateOnIntegerOverflow=off
  Abs1 : Abs  SaturateOnIntegerOverflow=off
  Complex to Real-Imag : ComplexToRealImag
  Delay : Delay  DelayLength=1
  Delay1 : Delay  DelayLength=1
  Max : MinMax  Function=max  Inputs=2
  Max1 : MinMax  Function=max  Inputs=2
  Real : Outport
  Imag : Outport  Port=2
  wires:
  Max/1 -> Real/1, Delay/1
  Delay/1 -> Max/1
  Max1/1 -> Imag/1, Delay1/1
  Delay1/1 -> Max1/1
  Complex to Real-Imag/2 -> Abs1/1
  Complex to Real-Imag/1 -> Abs/1
  In1/1 -> Complex to Real-Imag/1
  Abs/1 -> Max/2
  Abs1/1 -> Max1/2

== system OFDMmodel_synch/RX/Sincronizador de Trama/Metrica/IIR Recursivo/P(d)/Maximo3 ==
  In1 : Inport
  Abs : Abs  SaturateOnIntegerOverflow=off
  Abs1 : Abs  SaturateOnIntegerOverflow=off
  Complex to Real-Imag : ComplexToRealImag
  Delay : Delay  DelayLength=1
  Delay1 : Delay  DelayLength=1
  Max : MinMax  Function=max  Inputs=2
  Max1 : MinMax  Function=max  Inputs=2
  Real : Outport
  Imag : Outport  Port=2
  wires:
  Abs1/1 -> Max1/2
  Abs/1 -> Max/2
  In1/1 -> Complex to Real-Imag/1
  Complex to Real-Imag/1 -> Abs/1
  Complex to Real-Imag/2 -> Abs1/1
  Delay1/1 -> Max1/1
  Max1/1 -> Delay1/1, Imag/1
  Delay/1 -> Max/1
  Max/1 -> Delay/1, Real/1

== system OFDMmodel_synch/RX/Sincronizador de Trama/Metrica/IIR Recursivo/P(d)/Maximo4 ==
  Rx_in : Inport
  Abs : Abs  SaturateOnIntegerOverflow=off
  Abs1 : Abs  SaturateOnIntegerOverflow=off
  Complex to Real-Imag : ComplexToRealImag
  Delay : Delay  DelayLength=1
  Delay1 : Delay  DelayLength=1
  Max : MinMax  Function=max  Inputs=2
  Max1 : MinMax  Function=max  Inputs=2
  Real : Outport
  Imag : Outport  Port=2
  wires:
  Abs1/1 -> Max1/2
  Abs/1 -> Max/2
  Rx_in/1 -> Complex to Real-Imag/1
  Complex to Real-Imag/1 -> Abs/1
  Complex to Real-Imag/2 -> Abs1/1
  Delay1/1 -> Max1/1
  Max1/1 -> Delay1/1, Imag/1
  Delay/1 -> Max/1
  Max/1 -> Delay/1, Real/1

== system OFDMmodel_synch/RX/Sincronizador de Trama/Metrica/IIR Recursivo_Normalize/P(d)/Maximo ==
  In1 : Inport
  Abs : Abs  SaturateOnIntegerOverflow=off
  Abs1 : Abs  SaturateOnIntegerOverflow=off
  Complex to Real-Imag : ComplexToRealImag
  Delay : Delay  DelayLength=1
  Delay1 : Delay  DelayLength=1
  Max : MinMax  Function=max  Inputs=2
  Max1 : MinMax  Function=max  Inputs=2
  Real : Outport
  Imag : Outport  Port=2
  wires:
  Abs1/1 -> Max1/2
  Abs/1 -> Max/2
  In1/1 -> Complex to Real-Imag/1
  Complex to Real-Imag/1 -> Abs/1
  Complex to Real-Imag/2 -> Abs1/1
  Delay1/1 -> Max1/1
  Max1/1 -> Delay1/1, Imag/1
  Delay/1 -> Max/1
  Max/1 -> Delay/1, Real/1

== system OFDMmodel_synch/RX/Sincronizador de Trama/Metrica/IIR Recursivo_Normalize/P(d)/Maximo1 ==
  In1 : Inport
  Abs : Abs  SaturateOnIntegerOverflow=off
  Abs1 : Abs  SaturateOnIntegerOverflow=off
  Complex to Real-Imag : ComplexToRealImag
  Delay : Delay  DelayLength=1
  Delay1 : Delay  DelayLength=1
  Max : MinMax  Function=max  Inputs=2
  Max1 : MinMax  Function=max  Inputs=2
  Real : Outport
  Imag : Outport  Port=2
  wires:
  Max/1 -> Real/1, Delay/1
  Delay/1 -> Max/1
  Max1/1 -> Imag/1, Delay1/1
  Delay1/1 -> Max1/1
  Complex to Real-Imag/2 -> Abs1/1
  Complex to Real-Imag/1 -> Abs/1
  In1/1 -> Complex to Real-Imag/1
  Abs/1 -> Max/2
  Abs1/1 -> Max1/2

== system OFDMmodel_synch/RX/Sincronizador de Trama/Metrica/IIR Recursivo_Normalize/P(d)/Maximo2 ==
  In1 : Inport
  Abs : Abs  SaturateOnIntegerOverflow=off
  Abs1 : Abs  SaturateOnIntegerOverflow=off
  Complex to Real-Imag : ComplexToRealImag
  Delay : Delay  DelayLength=1
  Delay1 : Delay  DelayLength=1
  Max : MinMax  Function=max  Inputs=2
  Max1 : MinMax  Function=max  Inputs=2
  Real : Outport
  Imag : Outport  Port=2
  wires:
  Abs1/1 -> Max1/2
  Abs/1 -> Max/2
  In1/1 -> Complex to Real-Imag/1
  Complex to Real-Imag/1 -> Abs/1
  Complex to Real-Imag/2 -> Abs1/1
  Delay1/1 -> Max1/1
  Max1/1 -> Delay1/1, Imag/1
  Delay/1 -> Max/1
  Max/1 -> Delay/1, Real/1

== system OFDMmodel_synch/RX/Sincronizador de Trama/Metrica/IIR Recursivo_Normalize/P(d)/Maximo3 ==
  In1 : Inport
  Abs : Abs  SaturateOnIntegerOverflow=off
  Abs1 : Abs  SaturateOnIntegerOverflow=off
  Complex to Real-Imag : ComplexToRealImag
  Delay : Delay  DelayLength=1
  Delay1 : Delay  DelayLength=1
  Max : MinMax  Function=max  Inputs=2
  Max1 : MinMax  Function=max  Inputs=2
  Real : Outport
  Imag : Outport  Port=2
  wires:
  Max/1 -> Real/1, Delay/1
  Delay/1 -> Max/1
  Max1/1 -> Imag/1, Delay1/1
  Delay1/1 -> Max1/1
  Complex to Real-Imag/2 -> Abs1/1
  Complex to Real-Imag/1 -> Abs/1
  In1/1 -> Complex to Real-Imag/1
  Abs/1 -> Max/2
  Abs1/1 -> Max1/2

== system OFDMmodel_synch/RX/Sincronizador de Trama/Metrica/IIR Recursivo_Normalize/P(d)/Maximo4 ==
  Rx_in : Inport
  Abs : Abs  SaturateOnIntegerOverflow=off
  Abs1 : Abs  SaturateOnIntegerOverflow=off
  Complex to Real-Imag : ComplexToRealImag
  Delay : Delay  DelayLength=1
  Delay1 : Delay  DelayLength=1
  Max : MinMax  Function=max  Inputs=2
  Max1 : MinMax  Function=max  Inputs=2
  Real : Outport
  Imag : Outport  Port=2
  wires:
  Max/1 -> Real/1, Delay/1
  Delay/1 -> Max/1
  Max1/1 -> Imag/1, Delay1/1
  Delay1/1 -> Max1/1
  Complex to Real-Imag/2 -> Abs1/1
  Complex to Real-Imag/1 -> Abs/1
  Rx_in/1 -> Complex to Real-Imag/1
  Abs/1 -> Max/2
  Abs1/1 -> Max1/2

== matlab function OFDMmodel_synch/RX/MATLAB Function ==
  data: Matriz input; Q_matrix output; R_matrix output
function [Q_matrix, R_matrix] = qr_givens(Matriz)
% 
% block_len = length(rxSig);
% H = rand(block_len) + j*rand(block_len);
% rxSig = rand(block_len,1);
% 
% H_extendida = [H rxSig];
% 
% for k = 1:block_len
%     for i_qr = block_len-1:-1:k
%         j = k;
%         r = sqrt(abs(H_extendida(i_qr,j))^2 + abs(H_extendida(i_qr+1,j))^2);
%         if(r == 0)
%             c = 1;
%             s = 0;
%         else
%             c = conj(H_extendida(i_qr,j))/r;
%             s = conj(H_extendida(i_qr+1,j))/r;
%         end
% 
%         H_extendida(i_qr,j) = r;
%         H_extendida(i_qr+1,j) = 0;
% 
%         for j = k+1:block_len + 1
% 
%             aux = H_extendida(i_qr,j);
%             b = H_extendida(i_qr+1,j);
% 
%             H_extendida(i_qr,j) = c*aux + s*b;
%             H_extendida(i_qr+1,j) = -conj(s)*aux + conj(c)*b;
%         end
%     end
% end
% 
% R_matrix = H_extendida(1:block_len,1:end-1);
% Qh_y = H_extendida(:,end);
 
[Q_matrix, R_matrix] = qr(Matriz);

== matlab function OFDMmodel_synch/RX/MATLAB Function1 ==
  data: R input; x_est output; y_h input
function x_est = sic(R,y_h)

x_est = y_h;
